simulink model "openloop"  (R2022b)
settings: Solver=FixedStepAuto  StartTime=0.0  StopTime=0.16  RelTol=1e-3
libraries: simulink x1
settings Model: Creator=15403  LastModifiedBy=15403
settings OptimizationCC: DefaultParameterBehavior=Inlined  EnhancedBackFolding=on  PassReuseOutputArgsAs=Individual arguments  ZeroExternalMemoryAtStartup=off  ZeroInternalMemoryAtStartup=off  OptimizeBlockOrder=speed  DifferentSizesBufferReuse=on  OptimizationCustomize=off  EfficientTunableParamExpr=on
settings DebuggingCC: ParameterTunabilityLossMsg=error
settings HardwareCC: ProdBitPerPointer=32  ProdBitPerSizeT=32  ProdBitPerPtrDiffT=32  ProdLargestAtomicInteger=Long  ProdLargestAtomicFloat=Double  ProdWordSize=32  ProdHWDeviceType=ARM Compatible->ARM Cortex-M
settings SFSimCC: MATLABDynamicMemAlloc=off
settings RTWCC: Description=Embedded Coder  SystemTargetFile=ert.tlc  GenCodeOnly=on  PackageGeneratedCodeAndArtifacts=on  TemplateMakefile=ert_default_tmf  GenerateReport=on  LaunchReport=on
settings CodeAppCC: ForceParamTrailComments=on  IgnoreCustomStorageClasses=off  OperatorAnnotations=on  SimulinkDataObjDesc=on  SFDataObjDesc=on  InsertBlockDesc=on
settings ERTTargetCC: TargetLangStandard=C99 (ISO)  GenerateSampleERTMain=on  SupportContinuousTime=on  InlinedParameterPlacement=NonHierarchical  ERTCustomFileTemplate=example_file_process.tlc

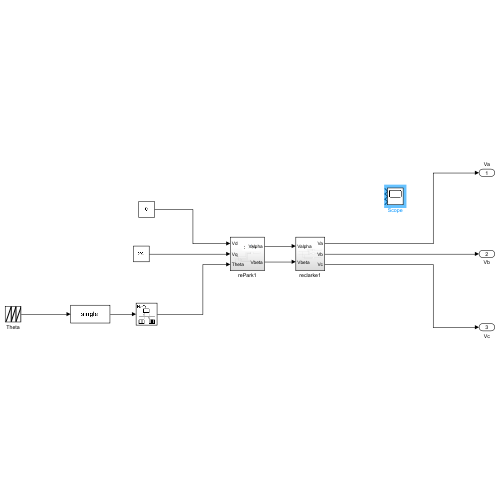
[thumbnail: Simulink's stored preview of the top-level diagram]
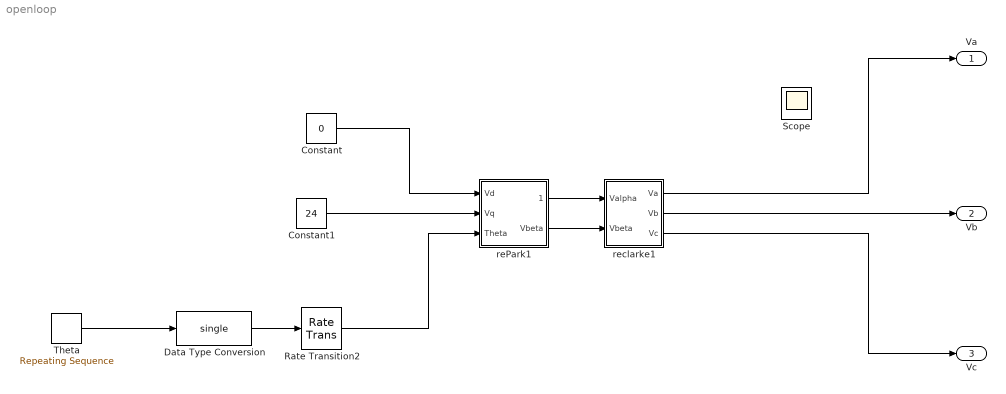
== system openloop ==
  Constant : Constant  Value=0
  Constant1 : Constant  Value=24
  Data Type Conversion : DataTypeConversion  OutDataTypeStr=single  SaturateOnIntegerOverflow=off  RndMeth=Floor
  Rate Transition2 : RateTransition
  Scope : Scope  NumInputPorts=3
  Theta : simulink/Sources/Repeating Sequence  rep_seq_t=[0 0.12]  rep_seq_y=[0 360]
  rePark1 : Subsystem
  reclarke1 : Subsystem
  Va : Outport
  Vb : Outport  Port=2
  Vc : Outport  Port=3
  wires:
  Data Type Conversion/1 -> Rate Transition2/1
  Rate Transition2/1 -> rePark1/3(Theta)
  reclarke1/2(Vb) -> Vb/1
  rePark1/1(Valpha) -> reclarke1/1(Valpha)
  Constant/1 -> rePark1/1(Vd)
  Theta/1 -> Data Type Conversion/1
  Constant1/1 -> rePark1/2(Vq)
  rePark1/2(Vbeta) -> reclarke1/2(Vbeta)
  reclarke1/1(Va) -> Va/1
  reclarke1/3(Vc) -> Vc/1

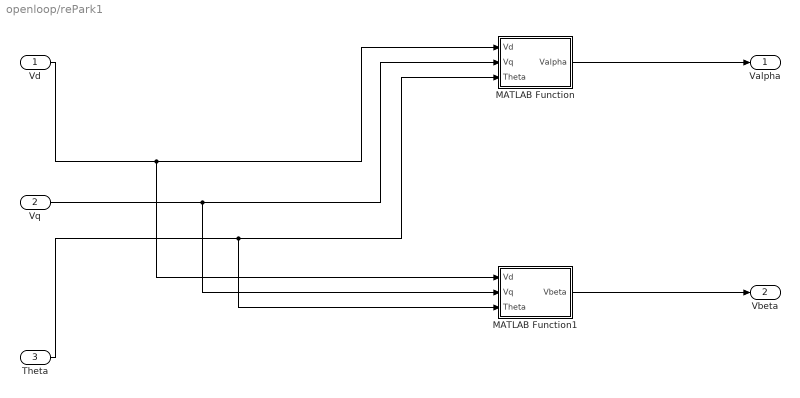
== system openloop/rePark1 ==
  Vd : Inport
  Vq : Inport  Port=2
  Theta : Inport  Port=3
  MATLAB Function : MATLAB Function  TreatAsAtomicUnit=on
  MATLAB Function1 : MATLAB Function  TreatAsAtomicUnit=on
  Valpha : Outport
  Vbeta : Outport  Port=2
  wires:
  Theta/1 -> MATLAB Function1/3(Theta), MATLAB Function/3(Theta)
  MATLAB Function1/1(Vbeta) -> Vbeta/1
  Vq/1 -> MATLAB Function1/2(Vq), MATLAB Function/2(Vq)
  Vd/1 -> MATLAB Function1/1(Vd), MATLAB Function/1(Vd)
  MATLAB Function/1(Valpha) -> Valpha/1

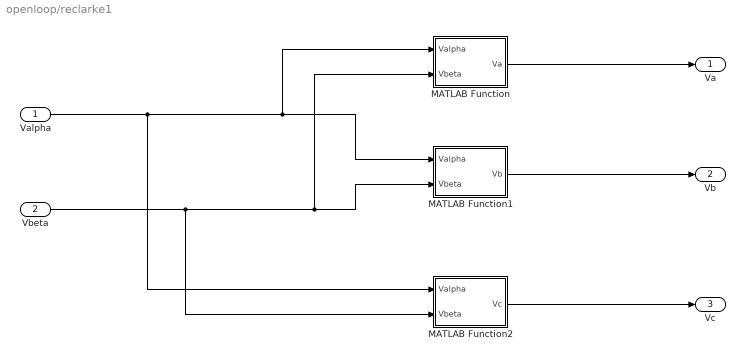
== system openloop/reclarke1 ==
  Valpha : Inport
  Vbeta : Inport  Port=2
  MATLAB Function : MATLAB Function  TreatAsAtomicUnit=on
  MATLAB Function1 : MATLAB Function  TreatAsAtomicUnit=on
  MATLAB Function2 : MATLAB Function  TreatAsAtomicUnit=on
  Va : Outport
  Vb : Outport  Port=2
  Vc : Outport  Port=3
  wires:
  Valpha/1 -> MATLAB Function2/1(Valpha), MATLAB Function/1(Valpha), MATLAB Function1/1(Valpha)
  MATLAB Function1/1(Vb) -> Vb/1
  Vbeta/1 -> MATLAB Function2/2(Vbeta), MATLAB Function/2(Vbeta), MATLAB Function1/2(Vbeta)
  MATLAB Function/1(Va) -> Va/1
  MATLAB Function2/1(Vc) -> Vc/1

== matlab function openloop/rePark1/MATLAB Function1 ==
  data: Vd input; Vbeta output; Vq input; Theta input
function Vbeta = fcn(Vd, Vq, Theta)

Vbeta = Vq * cosd(Theta) + Vd * sind(Theta);

== matlab function openloop/reclarke1/MATLAB Function ==
  data: Valpha input; Va output; Vbeta input
function Va = fcn(Valpha, Vbeta)

Va = Valpha;

== matlab function openloop/reclarke1/MATLAB Function1 ==
  data: Valpha input; Vb output; Vbeta input
function Vb = fcn(Valpha, Vbeta)

Vb = -Valpha * sind(30) + Vbeta * cosd(30);

== matlab function openloop/reclarke1/MATLAB Function2 ==
  data: Valpha input; Vc output; Vbeta input
function Vc = fcn(Valpha, Vbeta)

Vc = -Valpha * sind(30) - Vbeta * cosd(30);

== matlab function openloop/rePark1/MATLAB Function ==
  data: Vd input; Valpha output; Vq input; Theta input
function Valpha = fcn(Vd, Vq, Theta)

Valpha = -Vq * sind(Theta) + Vd * cosd(Theta);
